simulink model "gantry_center_laser"  (R2025b)
settings: Solver=FixedStepDiscrete  StartTime=0.0  StopTime=inf  FixedStep=0.05  RelTol=1e-3  EnableMultiTasking=on
libraries: raspberrypiBasiclib x5, simulink x5, raspberrypiNetworklib x1
settings Model: Creator=jeets  LastModifiedBy=jeets
settings SolverCC: PositivePriorityOrder=on
settings OptimizationCC: EnhancedBackFolding=on  PassReuseOutputArgsAs=Individual arguments  ZeroExternalMemoryAtStartup=off  ZeroInternalMemoryAtStartup=off  MaxStackSize=200000  OptimizeBlockOrder=speed  DifferentSizesBufferReuse=on  OptimizationCustomize=off  EfficientTunableParamExpr=on
settings DebuggingCC: ParameterTunabilityLossMsg=error
settings HardwareCC: ProdBitPerPointer=32.0  ProdBitPerSizeT=32.0  ProdBitPerPtrDiffT=32.0  ProdLargestAtomicInteger=Long  ProdLargestAtomicFloat=Double  ProdWordSize=32.0  ProdLongLongMode=on  ProdHWDeviceType=ARM Compatible->ARM Cortex-A (32-bit)
settings RTWCC: SystemTargetFile=ert.tlc  HardwareBoard=Raspberry Pi  TLCOptions="-aInlineSetEventsForThisBaseRateFcn=TLC_FALSE -aSuppressMultiTaskScheduler=TLC_FALSE  -aRateBasedStepFcn=0"  TemplateMakefile=ert_default_tmf  Toolchain=GNU GCC Embedded Linux  BuildConfiguration=Faster Runs  Description=Embedded Coder
settings CodeAppCC: ForceParamTrailComments=on  IgnoreCustomStorageClasses=off  OperatorAnnotations=on  SimulinkDataObjDesc=on  SFDataObjDesc=on  InsertBlockDesc=on
settings ERTTargetCC: ExtModeTransport=2.0  ExtModeStaticAlloc=on  ExtModeMexFile=ext_xcp  ExtModeIntrfLevel=Level2 - Open  InlinedParameterPlacement=Hierarchical  CodeReplacementLibrary=ARM Cortex-A CMSIS  SupportVariableSizeSignals=on

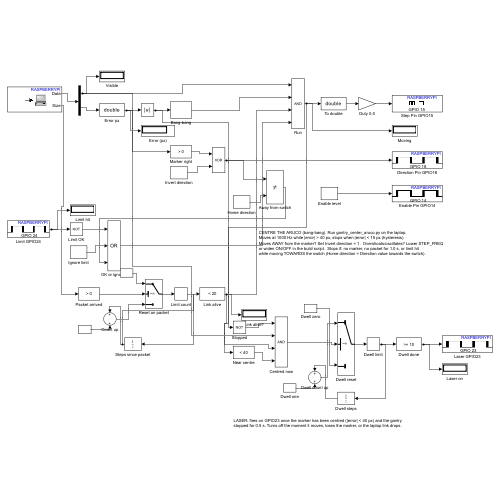
[thumbnail: Simulink's stored preview of the top-level diagram]
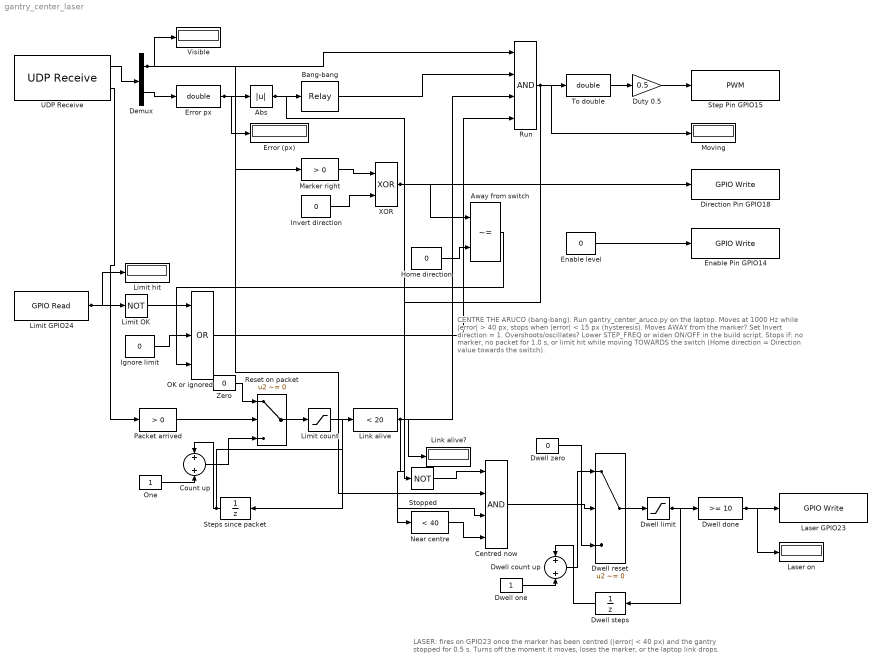
== system gantry_center_laser ==
  note: CENTRE THE ARUCO (bang-bang). Run gantry_center_aruco.py on the laptop.
      | Moves at 1000 Hz while |error| > 40 px, stops when |error| < 15 px (hysteresis).
      | Moves AWAY from the marker? Set Invert direction = 1.  Overshoots/oscillates? Lower STEP_FREQ
      | or widen ON/OFF in the build script.  Stops if: no marker, no packet for 1.0 s, or limit hit
      | while moving TOWARDS the switch (Home direction = Direction value towards the switch).
  note: LASER: fires on GPIO23 once the marker has been centred (|error| < 40 px) and the gantry
      | stopped for 0.5 s. Turns off the moment it moves, loses the marker, or the laptop link drops.
  Abs : Abs  SaturateOnIntegerOverflow=off
  Away from switch : RelationalOperator  Operator=~=  OutDataTypeStr=boolean  RndMeth=Simplest  InputSameDT=off
  Bang-bang : Relay  OnSwitchValue=40  OffSwitchValue=15
  Centred now : Logic  Inputs=4  AllPortsSameDT=off  OutDataTypeStr=boolean
  Count up : Sum
  Demux : Demux  Outputs=2
  Direction Pin GPIO18 : raspberrypiBasiclib/GPIO Write  BoardProperty=Pi 3 Model B+  gpio=18  blockPlatform=Raspberry Pi  PinNumber=17  board=[]  direction=[]
  Duty 0.5 : Gain  Gain=0.5
  Dwell count up : Sum
  Dwell done : simulink/Logic and Bit Operations/Compare To Constant  relop=>=  const=10  OutDataTypeStr=boolean
  Dwell limit : Saturate  UpperLimit=1000  LowerLimit=0
  Dwell one : Constant
  Dwell reset : Switch  Criteria=u2 ~= 0  SaturateOnIntegerOverflow=off  InputSameDT=off
  Dwell steps : UnitDelay  SampleTime=0.05  HasFrameUpgradeWarning=on
  Dwell zero : Constant  Value=0
  Enable Pin GPIO14 : raspberrypiBasiclib/GPIO Write  BoardProperty=Pi 3 Model B+  gpio=14  blockPlatform=Raspberry Pi  PinNumber=17  board=[]  direction=[]
  Enable level : Constant  Value=0  OutDataTypeStr=boolean
  Error (px) : Display
  Error px : DataTypeConversion  OutDataTypeStr=double  SaturateOnIntegerOverflow=off  RndMeth=Floor
  Home direction : Constant  Value=0
  Ignore limit : Constant  Value=0
  Invert direction : Constant  Value=0
  Laser GPIO23 : raspberrypiBasiclib/GPIO Write  BoardProperty=Pi 3 Model B+  gpio=23  blockPlatform=Raspberry Pi  PinNumber=17  board=[]  direction=[]
  Laser on : Display
  Limit GPIO24 : raspberrypiBasiclib/GPIO Read  BoardProperty=Pi 3 Model B+  gpio=24  SampleTime=0.05  blockPlatform=Raspberry Pi  PinNumber=4  board=[]  direction=[]  internalResistor=[]
  Limit OK : Logic  Operator=NOT  AllPortsSameDT=off  OutDataTypeStr=boolean
  Limit count : Saturate  UpperLimit=1000  LowerLimit=0
  Limit hit : Display
  Link alive : simulink/Logic and Bit Operations/Compare To Constant  relop=<  const=20  OutDataTypeStr=boolean
  Link alive? : Display
  Marker right : simulink/Logic and Bit Operations/Compare To Zero  relop=>  OutDataTypeStr=boolean
  Moving : Display
  Near centre : simulink/Logic and Bit Operations/Compare To Constant  relop=<  const=40  OutDataTypeStr=boolean
  OK or ignored : Logic  Operator=OR  Inputs=3  AllPortsSameDT=off  OutDataTypeStr=boolean
  One : Constant
  Packet arrived : simulink/Logic and Bit Operations/Compare To Zero  relop=>  OutDataTypeStr=boolean
  Reset on packet : Switch  Criteria=u2 ~= 0  SaturateOnIntegerOverflow=off  InputSameDT=off
  Run : Logic  Inputs=4  AllPortsSameDT=off  OutDataTypeStr=boolean
  Step Pin GPIO15 : raspberrypiBasiclib/PWM  board=Pi 3 Model B+  Pin_=15  Frequency=1000  blockPlatform=Raspberry Pi
  Steps since packet : UnitDelay  InitialCondition=20  SampleTime=0.05  HasFrameUpgradeWarning=on
  Stopped : Logic  Operator=NOT  AllPortsSameDT=off  OutDataTypeStr=boolean
  To double : DataTypeConversion  OutDataTypeStr=double  SaturateOnIntegerOverflow=off  RndMeth=Floor
  UDP Receive : raspberrypiNetworklib/UDP Receive  localURL='0.0.0.0'  localPort=50001  remoteURL='0.0.0.0'  remotePort=-1  recvBufferSize=8192  signalDatatype=int16  dims=2  isVarSize=off  showBlockingTime=off  blockingTime=0  sampletime=0.05  blockPlatform=Raspberry Pi
  Visible : Display
  XOR : Logic  Operator=XOR  AllPortsSameDT=off  OutDataTypeStr=boolean
  Zero : Constant  Value=0
  wires:
  UDP Receive/1 -> Demux/1
  Demux/1 -> Run/1, Visible/1, Centred now/2
  Demux/2 -> Error px/1
  Error px/1 -> Abs/1, Error (px)/1, Marker right/1
  Abs/1 -> Bang-bang/1, Near centre/1
  Bang-bang/1 -> Run/2
  Link alive/1 -> Run/3, Link alive?/1, Centred now/3
  OK or ignored/1 -> Run/4
  Run/1 -> To double/1, Moving/1, Stopped/1
  To double/1 -> Duty 0.5/1
  Duty 0.5/1 -> Step Pin GPIO15/1
  Marker right/1 -> XOR/1
  Invert direction/1 -> XOR/2
  XOR/1 -> Direction Pin GPIO18/1, Away from switch/1
  Enable level/1 -> Enable Pin GPIO14/1
  Limit GPIO24/1 -> Limit OK/1, Limit hit/1
  Limit OK/1 -> OK or ignored/1
  Ignore limit/1 -> OK or ignored/2
  Home direction/1 -> Away from switch/2
  Away from switch/1 -> OK or ignored/3
  UDP Receive/2 -> Packet arrived/1
  Zero/1 -> Reset on packet/1
  Packet arrived/1 -> Reset on packet/2
  Count up/1 -> Reset on packet/3
  Reset on packet/1 -> Limit count/1
  Limit count/1 -> Steps since packet/1
  Steps since packet/1 -> Count up/1, Link alive/1
  One/1 -> Count up/2
  Stopped/1 -> Centred now/1
  Near centre/1 -> Centred now/4
  Dwell count up/1 -> Dwell reset/1
  Centred now/1 -> Dwell reset/2
  Dwell zero/1 -> Dwell reset/3
  Dwell reset/1 -> Dwell limit/1
  Dwell limit/1 -> Dwell steps/1, Dwell done/1
  Dwell steps/1 -> Dwell count up/1
  Dwell one/1 -> Dwell count up/2
  Dwell done/1 -> Laser GPIO23/1, Laser on/1
